simulink model "snap_adc5g_spec"  (R2019a)
settings: Solver=VariableStepDiscrete  StartTime=0.0  StopTime=10.0  RelTol=1e-3
undefined symbols (not defined in the file): pfb_coeff_gen_calc
libraries: xbsIndex_r4 x13965, casper_library_misc x80, casper_library_delays x43, xps_library x5, xbsReplacements_r4 x2, casper_library_communications x1
(part 75 of 152)

== system snap_adc5g_spec/fft_wideband_real/fft_biplex_real_4x/biplex_core/fft_stage_11/butterfly_direct/twiddle ==
  ai : Inport
  bi : Inport  Port=2
  sync_in : Inport  Port=3
  bus_convert : Subsystem  AncestorBlock=casper_library_bus/bus_convert  mask(bus_convert){n_bits_in=repmat(input_bit_width+coeff_bit_width+1, 1, n_inputs), bin_pt_in=(bin_pt_in+coeff_bit_width-1), cmplx=on, n_bits_out=input_bit_width+1, bin_pt_out=bin_pt_in, quantization=2, overflow=0, csp_latency=conv_latency, of=off, misc=on}
      mask prompts: n_bits_in "input bit widths"; bin_pt_in "input binary points"; cmplx "input complex"; n_bits_out "output bit widths"; bin_pt_out "output binary points"; quantization "quantization strategy (Truncate=0, Round  (unbiased: +/- Inf)=1, Round (unbiased: Even Values)=2)"; overflow "overflow strategy (Wrap=0, Saturate=1, Flag as error=2)"; csp_latency "latency"; of "overflow indication"; misc "misc support"
      mask help: Convert components of busses
      mask init: same as snap_adc5g_spec/fft_wideband_real/fft_direct/butterfly0_0/bus_convert
  bus_create : Subsystem  AncestorBlock=casper_library_flow_control/bus_create  mask(bus_create){inputNum=3}
      mask prompts: inputNum "Number of inputs:"
      mask init:
      | bus_create_init(gcb,...
      |     'inputNum', inputNum);
  bus_expand : Subsystem  AncestorBlock=casper_library_flow_control/bus_expand  mask(bus_expand){mode=divisions of arbitrary size, outputNum=1, outputWidth=[n_inputs*input_bit_width*2, 1+(n_inputs*input_bit_width*2)], outputBinaryPt=[0 0], outputArithmeticType=[0 0], show_format=off, outputToWorkspace=off, variablePrefix=out, outputToModelAsWell=on}
      mask prompts: outputNum "Number of outputs:"; outputWidth "Output width [msb ... lsb]:"; outputBinaryPt "Output binary point position [msb ... lsb]:"; outputArithmeticType "Output arithmetic type (ufix=0, fix=1, bool=2) [msb ... lsb]:"; show_format "Print format string?"; outputToWorkspace "Output to workspace?"; variablePrefix "Variable name prefix:"; outputToModelAsWell "Output to model as well?"
      mask help:
      | Expands a 'bus' made using a bus_create or Xilinx
      | concat block.
      | The input will be divided into the specified number
      | of outputs with the specified arithmetic types.
      | Divisions are made from most significant bit.
      mask init: same as snap_adc5g_spec/ss_adc/ctrl_split
      settings: AttributesFormatString=2 outputs
      mask TypeOptions mode: divisions of equal size | divisions of arbitrary size
      mask Callback mode: bus_expand_callback();
      mask Callback outputWidth: bus_expand_callback();
      mask Callback outputToWorkspace: bus_expand_callback();
  bus_expand1 : Subsystem  AncestorBlock=casper_library_flow_control/bus_expand  mask(bus_expand){mode=divisions of arbitrary size, outputNum=1, outputWidth=[1 72], outputBinaryPt=[0 0], outputArithmeticType=[2 0], show_format=off, outputToWorkspace=off, variablePrefix=out, outputToModelAsWell=on}
      mask prompts: outputNum "Number of outputs:"; outputWidth "Output width [msb ... lsb]:"; outputBinaryPt "Output binary point position [msb ... lsb]:"; outputArithmeticType "Output arithmetic type (ufix=0, fix=1, bool=2) [msb ... lsb]:"; show_format "Print format string?"; outputToWorkspace "Output to workspace?"; variablePrefix "Variable name prefix:"; outputToModelAsWell "Output to model as well?"
      mask help:
      | Expands a 'bus' made using a bus_create or Xilinx
      | concat block.
      | The input will be divided into the specified number
      | of outputs with the specified arithmetic types.
      | Divisions are made from most significant bit.
      mask init: same as snap_adc5g_spec/ss_adc/ctrl_split
      settings: AttributesFormatString=2 outputs
      mask TypeOptions mode: divisions of equal size | divisions of arbitrary size
      mask Callback mode: bus_expand_callback();
      mask Callback outputWidth: bus_expand_callback();
      mask Callback outputToWorkspace: bus_expand_callback();
  bus_mult : Subsystem  AncestorBlock=casper_library_bus/bus_mult  mask(bus_mult){n_bits_a=coeff_bit_width, bin_pt_a=coeff_bit_width-1, type_a=1, cmplx_a=on, n_bits_b=[18 18], bin_pt_b=bin_pt_in, type_b=1, cmplx_b=on, misc=on, floating_point=off, float_type=single, input_vec_a=1, input_vec_b=1, frac_width=24, exp_width=8, n_bits_out=input_bit_width+coeff_bit_width+1, bin_pt_out=(bin_pt_in+coeff_bit_width-1), type_out=1, quantization=0, overflow=0, mult_latency=mult_latency, add_latency=add_latency, conv_latency=0, max_fanout=max_fanout, fan_latency=2, multiplier_implementation=behavioral HDL, pipeline_cmult_en=off, pipeline_latency=0}
      mask prompts: n_bits_a "a input bit widths"; bin_pt_a "a input binary points"; type_a "a input type (Unsigned=0, Signed=1)"; cmplx_a "a input complex"; n_bits_b "b input bit widths"; bin_pt_b "b input binary points"; type_b "b input type (Unsigned=0, Signed=1)"; cmplx_b "b input complex"; misc "misc support"; floating_point "floating point"; float_type "float type"; input_vec_a "a input vector in bus"; input_vec_b "b input vector in bus"; frac_width "fraction width"; exp_width "exponent width"; n_bits_out "output bit widths"; bin_pt_out "output binary points"; type_out "output type (Unsigned=0, Signed=1)"; quantization "quantization strategy (Truncate=0, Round  (unbiased: +/- Inf)=1)"; overflow "overflow strategy (Wrap=0, Saturate=1, Flag as error=2)"; mult_latency "multiplier latency"; add_latency "adder latency"; conv_latency "convert latency"; max_fanout "limit fanout to ?"; fan_latency "fanout register latency"; multiplier_implementation "multiplier implementation"; pipeline_cmult_en "pipeline complex mult"; pipeline_latency "pipeline latency"
      mask help: Multiply components of two busses
      mask init: same as snap_adc5g_spec/fft_wideband_real/fft_direct/butterfly0_0/twiddle/bus_mult
      mask Callback floating_point:
      | onoff = get_param(gcb, 'floating_point');
      | if strcmp(onoff,'on')
      |     enable_fixpt = 'off';
      |     set_param_state(gcb, 'float_type', 'on')
      | 
      |     set_param_state(gcb, 'input_vec_a', 'on')
      |     set_param_state(gcb, 'input_vec_b', 'on')
      | 
      |     f_type = get_param(gcb, 'float_type');
      |     if strcmp(f_type,'custom')
      |         set_param_state(gcb, 'exp_width', 'on')
      |         set_param_state(gcb, 'frac_width', 'on')
      |     else
      |         set_param_state(gcb, 'exp_width', 'off')
      |         set_param_state(gcb, 'frac_width', 'off')
      |     end
      | 
      | else
      |     enable_fixpt = 'on';
      |     set_param_state(gcb, 'float_type', 'off')
      |     set_param_state(gcb, 'exp_width', 'off')
      |     set_param_state(gcb, 'frac_width', 'off')
      |     set_param_state(gcb, 'input_vec_a', 'off')
      |     set_param_state(gcb, 'input_vec_b', 'off')
      | end
      | 
      | set_param_state(gcb, 'n_bits_a', enable_fixpt)
      | set_param_state(gcb, 'bin_pt_a', enable_fixpt)
      | set_param_state(gcb, 'type_a', enable_fixpt)
      | set_param_state(gcb, 'n_bits_b', enable_fixpt)
      | set_param_state(gcb, 'bin_pt_b', enable_fixpt)
      | set_param_state(gcb, 'type_b', enable_fixpt)
      | 
      | set_param_state(gcb, 'n_bits_out', enable_fixpt)
      | set_param_state(gcb, 'bin_pt_out', enable_fixpt)
      | set_param_state(gcb, 'type_out', enable_fixpt)
      | set_param_state(gcb, 'quantization', enable_fixpt)
      | set_param_state(gcb, 'overflow', enable_fixpt)
      mask TypeOptions float_type: single | custom
      mask Callback float_type:
      | f_type = get_param(gcb, 'float_type');
      | if strcmp(f_type,'custom')
      |     set_param_state(gcb, 'exp_width', 'on')
      |     set_param_state(gcb, 'frac_width', 'on')
      | else
      |     set_param_state(gcb, 'exp_width', 'off')
      |     set_param_state(gcb, 'frac_width', 'off')
      | end
      mask TypeOptions multiplier_implementation: behavioral HDL | standard core | embedded multiplier core
      mask Callback pipeline_cmult_en:
      | pipeline_en = get_param(gcb, 'pipeline_cmult_en');
      | if strcmp(pipeline_en,'on')
      | 
      |     set_param_state(gcb, 'pipeline_latency', 'on')
      | else
      |     set_param_state(gcb, 'pipeline_latency', 'off')
      | end
  coeff_gen : Subsystem  AncestorBlock=casper_library_ffts_twiddle_coeff_gen/coeff_gen  mask(coeff_gen){FFTSize=FFTSize, Coeffs=[0 1 2 3 4 5 6 7 8 9 10 11 12 13 14 15 16 17 18 19 20 21 22 23 24 25 26 27 28 29 30 31 32 33 34 35 36 37 38 39 40 41 42 43 44 45 46 47 48 49 50 51 52 53 54 55 56 57 58 59 60 61 62 63 64 65 66 67 68 69 70 71 72 73 74 75 76 77 78 79 80 81 82 83 84 85 86 87 88 89 90 91 92 93 94 95 96 97 98 99 100 101 102 103 104 105 106 107 108 109 110 111 112 113 114 115 116 117 118 119 120 121 122 123 124 125 126 127 128 129 130 131 132 133 134 135 136 137 138 139 140 141 142 143 144 145 146 147 148 149 150 151 152 153 154 155 156 157 158 159 160 161 162 163 164 165 166 167 168 169 170 171 172 173 174 175 176 177 178 179 180 181 182 183 184 185 186 187 188 189 190 191 192 193 194 195 196 197 198 199 200 201 202 203 204 205 206 207 208 209 210 211 212 213 214 215 216 217 218 219 220 221 222 223 224 225 226 227 228 229 230 231 232 233 234 235 236 237 238 239 240 241 242 243 244 245 246 247 248 249 250 251 252 253 254 255 256 257 258 259 260 261 262 263 264 265 266 267 268 269 270 271 272 273 274 275 276 277 278 279 280 281 282 283 284 285 286 287 288 289 290 291 292 293 294 295 296 297 298 299 300 301 302 303 304 305 306 307 308 309 310 311 312 313 314 315 316 317 318 319 320 321 322 323 324 325 326 327 328 329 330 331 332 333 334 335 336 337 338 339 340 341 342 343 344 345 346 347 348 349 350 351 352 353 354 355 356 357 358 359 360 361 362 363 364 365 366 367 368 369 370 371 372 373 374 375 376 377 378 379 380 381 382 383 384 385 386 387 388 389 390 391 392 393 394 395 396 397 398 399 400 401 402 403 404 405 406 407 408 409 410 411 412 413 414 415 416 417 418 419 420 421 422 423 424 425 426 427 428 429 430 431 432 433 434 435 436 437 438 439 440 441 442 443 444 445 446 447 448 449 450 451 452 453 454 455 456 457 458 459 460 461 462 463 464 465 466 467 468 469 470 471 472 473 474 475 476 477 478 479 480 481 482 483 484 485 486 487 488 489 490 491 492 493 494 495 496 497 498 499 500 501 502 503 504 505 506 507 508 509 510 511 512 513 514 515 516 517 518 519 520 521 522 523 524 525 526 527 528 529 530 531 532 533 534 535 536 537 538 539 540 541 542 543 544 545 546 547 548 549 550 551 552 553 554 555 556 557 558 559 560 561 562 563 564 565 566 567 568 569 570 571 572 573 574 575 576 577 578 579 580 581 582 583 584 585 586 587 588 589 590 591 592 593 594 595 596 597 598 599 600 601 602 603 604 605 606 607 608 609 610 611 612 613 614 615 616 617 618 619 620 621 622 623 624 625 626 627 628 629 630 631 632 633 634 635 636 637 638 639 640 641 642 643 644 645 646 647 648 649 650 651 652 653 654 655 656 657 658 659 660 661 662 663 664 665 666 667 668 669 670 671 672 673 674 675 676 677 678 679 680 681 682 683 684 685 686 687 688 689 690 691 692 693 694 695 696 697 698 699 700 701 702 703 704 705 706 707 708 709 710 711 712 713 714 715 716 717 718 719 720 721 722 723 724 725 726 727 728 729 730 731 732 733 734 735 736 737 738 739 740 741 742 743 744 745 746 747 748 749 750 751 752 753 754 755 756 757 758 759 760 761 762 763 764 765 766 767 768 769 770 771 772 773 774 775 776 777 778 779 780 781 782 783 784 785 786 787 788 789 790 791 792 793 794 795 796 797 798 799 800 801 802 803 804 805 806 807 808 809 810 811 812 813 814 815 816 817 818 819 820 821 822 823 824 825 826 827 828 829 830 831 832 833 834 835 836 837 838 839 840 841 842 843 844 845 846 847 848 849 850 851 852 853 854 855 856 857 858 859 860 861 862 863 864 865 866 867 868 869 870 871 872 873 874 875 876 877 878 879 880 881 882 883 884 885 886 887 888 889 890 891 892 893 894 895 896 897 898 899 900 901 902 903 904 905 906 907 908 909 910 911 912 913 914 915 916 917 918 919 920 921 922 923 924 925 926 927 928 929 930 931 932 933 934 935 936 937 938 939 940 941 942 943 944 945 946 947 948 949 950 951 952 953 954 955 956 957 958 959 960 961 962 963 964 965 966 967 968 969 970 971 972 973 974 975 976 977 978 979 980 981 982 983 984 985 986 987 988 989 990 991 992 993 994 995 996 997 998 999 1000 1001 1002 1003 1004 1005 1006 1007 1008 1009 1010 1011 1012 1013 1014 1015 1016 1017 1018 1019 1020 1021 1022 1023], coeff_bit_width=coeff_bit_width, StepPeriod=StepPeriod, async=off, misc=on, floating_point=off, float_type=single, exp_width=8, frac_width=24, bram_latency=bram_latency, mult_latency=mult_latency, add_latency=add_latency, conv_latency=conv_latency, coeffs_bit_limit=coeffs_bit_limit, coeff_sharing=on, coeff_decimation=on, coeff_generation=off, cal_bits=cal_bits, n_bits_rotation=n_bits_rotation, quantization=Round  (unbiased: Even Values)}
      mask prompts: FFTSize "fft size (2^?)"; Coeffs "Coefficients"; coeff_bit_width "Coefficient Bit Width:"; StepPeriod "Step Period: (2^?)"; async "asynchronous operation"; misc "misc port"; floating_point "floating point"; exp_width "exponential width"; frac_width "fractional width"; bram_latency "BRAM latency"; mult_latency "Multiplier latency"; add_latency "Adder latency"; conv_latency "Convert latency"; coeffs_bit_limit "Number bits above which to store stage's coefficients in BRAM (2^? bits)"; coeff_sharing "BRAM sharing in coeff storage"; coeff_decimation "Store a fraction of coeff factors where useful"; coeff_generation "Generate coeffs with multipliers where useful"; cal_bits "Number calibration locations when generating coeffs (2^?)"; n_bits_rotation "Rotation vector resolution"; quantization "Quantization strategy"
      mask help:
      | Generates a sequence of complex coefficients for use in generating twiddle
      | factors for FFTs.
      mask init: same as snap_adc5g_spec/fft_wideband_real/fft_direct/butterfly0_0/twiddle/coeff_gen
      settings: AttributesFormatString=1024 @ (18,17)
      mask Callback floating_point:
      | onoff = get_param(gcb, 'floating_point');
      | if strcmp(onoff,'on')
      |     enable_fixpt = 'off'
      |     set_param_state(gcb, 'float_type', 'on')
      | 
      |     f_type = get_param(gcb, 'float_type')
      |     if strcmp(f_type,'custom')
      |         set_param_state(gcb, 'exp_width', 'on')
      |         set_param_state(gcb, 'frac_width', 'on')
      |     else
      |         set_param_state(gcb, 'exp_width', 'off')
      |         set_param_state(gcb, 'frac_width', 'off')
      |     end
      | 
      | 
      | else
      |     enable_fixpt = 'on'
      |     set_param_state(gcb, 'float_type', 'off')
      |     set_param_state(gcb, 'exp_width', 'off')
      |     set_param_state(gcb, 'frac_width', 'off')
      | end
      mask TypeOptions float_type: single | custom
      mask Callback float_type:
      | f_type = get_param(gcb, 'float_type')
      | if strcmp(f_type,'custom')
      |     set_param_state(gcb, 'exp_width', 'on')
      |     set_param_state(gcb, 'frac_width', 'on')
      | else
      |     set_param_state(gcb, 'exp_width', 'off')
      |     set_param_state(gcb, 'frac_width', 'off')
      | end
      mask TypeOptions quantization: Truncate | Round  (unbiased: +/- Inf) | Round  (unbiased: Even Values)
      mask DialogControl ParameterTabVar0 Prompt: basic
      mask DialogControl ParameterTabVar01 Prompt: latency
      mask DialogControl ParameterTabVar012 Prompt: implementation
  ao : Outport
  bwo : Outport  Port=2
  sync_out : Outport  Port=3
  wires:
  bi/1 -> bus_create/1(in1)
  sync_in/1 -> bus_create/2(in2), coeff_gen/1(rst)
  ai/1 -> bus_create/3(in3)
  bus_create/1(bus_out) -> coeff_gen/2(misci)
  coeff_gen/2(misco) -> bus_expand/1(bus_in)
  coeff_gen/1(w) -> bus_mult/1(a)
  bus_expand/2(lsb_out1) -> bus_mult/3(misci)
  bus_expand/1(msb_out2) -> bus_mult/2(b)
  bus_mult/1(a*b) -> bus_convert/1(din)
  bus_mult/2(misco) -> bus_convert/2(misci)
  bus_convert/1(dout) -> bwo/1
  bus_convert/2(misco) -> bus_expand1/1(bus_in)
  bus_expand1/1(msb_out2) -> sync_out/1
  bus_expand1/2(lsb_out1) -> ao/1

== system snap_adc5g_spec/fft_wideband_real/fft_biplex_real_4x/biplex_core/fft_stage_11/delay0/din_expand ==
  bus_in : Inport
  reinterpret1 : xbsIndex_r4/Reinterpret  force_arith_type=on  arith_type=Unsigned  force_bin_pt=on  bin_pt=0  block_type=reinterpret
  reinterpret2 : xbsIndex_r4/Reinterpret  force_arith_type=on  arith_type=Unsigned  force_bin_pt=on  bin_pt=0  block_type=reinterpret
  slice1 : xbsIndex_r4/Slice  nbits=36  boolean_output=off  mode=Upper Bit Location + Width  bit1=-36  base1=MSB of Input  bit0=0  base0=LSB of Input  dbl_ovrd=off  block_type=slice
  slice2 : xbsIndex_r4/Slice  nbits=36  boolean_output=off  mode=Upper Bit Location + Width  bit1=0  base1=MSB of Input  bit0=0  base0=LSB of Input  dbl_ovrd=off  block_type=slice
  msb_out2 : Outport
  lsb_out1 : Outport  Port=2
  wires:
  bus_in/1 -> slice2/1, slice1/1
  slice2/1 -> reinterpret2/1
  reinterpret2/1 -> msb_out2/1
  slice1/1 -> reinterpret1/1
  reinterpret1/1 -> lsb_out1/1

== system snap_adc5g_spec/fft_wideband_real/fft_biplex_real_4x/biplex_core/fft_stage_11/delay0/dout_compress ==
  in1 : Inport
  in2 : Inport  Port=2
  concatenate : xbsIndex_r4/Concat  num_inputs=2  dbl_ovrd=off  block_type=concat
  reinterpret1 : xbsIndex_r4/Reinterpret  force_arith_type=on  arith_type=Unsigned  force_bin_pt=on  bin_pt=0  block_type=reinterpret
      settings: infoedit="Changes signal type without altering the binary representation.   You can changed the signal between signed and unsigned, and relocate the binary point.<br><br>Hardware notes: In hardware this block costs nothing.<br><br>Example:  Suppose the input is 6 bits wide, signed, with 2 fractional bits, and the output is forced to unsigned with 0 fractional bits.  Then an input of -2.0 (1110.00 in binary 2's complement) becomes an output of 56 (111000 in binary)."
  reinterpret2 : xbsIndex_r4/Reinterpret  force_arith_type=on  arith_type=Unsigned  force_bin_pt=on  bin_pt=0  block_type=reinterpret
      settings: infoedit="Changes signal type without altering the binary representation.   You can changed the signal between signed and unsigned, and relocate the binary point.<br><br>Hardware notes: In hardware this block costs nothing.<br><br>Example:  Suppose the input is 6 bits wide, signed, with 2 fractional bits, and the output is forced to unsigned with 0 fractional bits.  Then an input of -2.0 (1110.00 in binary 2's complement) becomes an output of 56 (111000 in binary)."
  bus_out : Outport
  wires:
  concatenate/1 -> bus_out/1
  in1/1 -> reinterpret1/1
  reinterpret1/1 -> concatenate/1
  in2/1 -> reinterpret2/1
  reinterpret2/1 -> concatenate/2

== system snap_adc5g_spec/fft_wideband_real/fft_biplex_real_4x/biplex_core/fft_stage_11/delay1/din_expand ==
  bus_in : Inport
  reinterpret1 : xbsIndex_r4/Reinterpret  force_arith_type=on  arith_type=Unsigned  force_bin_pt=on  bin_pt=0  block_type=reinterpret
  reinterpret2 : xbsIndex_r4/Reinterpret  force_arith_type=on  arith_type=Unsigned  force_bin_pt=on  bin_pt=0  block_type=reinterpret
  slice1 : xbsIndex_r4/Slice  nbits=36  boolean_output=off  mode=Upper Bit Location + Width  bit1=-36  base1=MSB of Input  bit0=0  base0=LSB of Input  dbl_ovrd=off  block_type=slice
  slice2 : xbsIndex_r4/Slice  nbits=36  boolean_output=off  mode=Upper Bit Location + Width  bit1=0  base1=MSB of Input  bit0=0  base0=LSB of Input  dbl_ovrd=off  block_type=slice
  msb_out2 : Outport
  lsb_out1 : Outport  Port=2
  wires:
  bus_in/1 -> slice2/1, slice1/1
  slice2/1 -> reinterpret2/1
  reinterpret2/1 -> msb_out2/1
  slice1/1 -> reinterpret1/1
  reinterpret1/1 -> lsb_out1/1

== system snap_adc5g_spec/fft_wideband_real/fft_biplex_real_4x/biplex_core/fft_stage_11/delay1/dout_compress ==
  in1 : Inport
  in2 : Inport  Port=2
  concatenate : xbsIndex_r4/Concat  num_inputs=2  dbl_ovrd=off  block_type=concat
  reinterpret1 : xbsIndex_r4/Reinterpret  force_arith_type=on  arith_type=Unsigned  force_bin_pt=on  bin_pt=0  block_type=reinterpret
      settings: infoedit="Changes signal type without altering the binary representation.   You can changed the signal between signed and unsigned, and relocate the binary point.<br><br>Hardware notes: In hardware this block costs nothing.<br><br>Example:  Suppose the input is 6 bits wide, signed, with 2 fractional bits, and the output is forced to unsigned with 0 fractional bits.  Then an input of -2.0 (1110.00 in binary 2's complement) becomes an output of 56 (111000 in binary)."
  reinterpret2 : xbsIndex_r4/Reinterpret  force_arith_type=on  arith_type=Unsigned  force_bin_pt=on  bin_pt=0  block_type=reinterpret
      settings: infoedit="Changes signal type without altering the binary representation.   You can changed the signal between signed and unsigned, and relocate the binary point.<br><br>Hardware notes: In hardware this block costs nothing.<br><br>Example:  Suppose the input is 6 bits wide, signed, with 2 fractional bits, and the output is forced to unsigned with 0 fractional bits.  Then an input of -2.0 (1110.00 in binary 2's complement) becomes an output of 56 (111000 in binary)."
  bus_out : Outport
  wires:
  concatenate/1 -> bus_out/1
  in1/1 -> reinterpret1/1
  reinterpret1/1 -> concatenate/1
  in2/1 -> reinterpret2/1
  reinterpret2/1 -> concatenate/2

== system snap_adc5g_spec/fft_wideband_real/fft_biplex_real_4x/biplex_core/fft_stage_2/butterfly_direct/bus_add ==
  a : Inport
  b : Inport  Port=2
  a_debus : Subsystem  AncestorBlock=casper_library_flow_control/bus_expand  mask(bus_expand){mode=divisions of arbitrary size, outputNum=1, outputWidth=[18  18  18  18], outputBinaryPt=[17  17  17  17], outputArithmeticType=[1  1  1  1], show_format=on, outputToWorkspace=off, variablePrefix=, outputToModelAsWell=on}
      mask prompts: outputNum "Number of outputs:"; outputWidth "Output width [msb ... lsb]:"; outputBinaryPt "Output binary point position [msb ... lsb]:"; outputArithmeticType "Output arithmetic type (ufix=0, fix=1, bool=2) [msb ... lsb]:"; show_format "Print format string?"; outputToWorkspace "Output to workspace?"; variablePrefix "Variable name prefix:"; outputToModelAsWell "Output to model as well?"
      mask help:
      | Expands a 'bus' made using a bus_create or Xilinx
      | concat block.
      | The input will be divided into the specified number
      | of outputs with the specified arithmetic types.
      | Divisions are made from most significant bit.
      mask init: same as snap_adc5g_spec/ss_adc/ctrl_split
      settings: AttributesFormatString=4 outputs: f18.17,f18.17,f18.17,f18.17,
      mask TypeOptions mode: divisions of equal size | divisions of arbitrary size
      mask Callback mode: bus_expand_callback();
      mask Callback outputWidth: bus_expand_callback();
      mask Callback outputToWorkspace: bus_expand_callback();
  addsub{1..4} (4 alike) : xbsIndex_r4/AddSub  mode=Addition  use_carryin=off  use_carryout=off  en=off  latency=1  precision=User Defined  arith_type="Signed  (2's comp)"  n_bits=19  bin_pt=17  quantization=Truncate  overflow=Wrap  use_behavioral_HDL=on  hw_selection=Fabric  pipelined=on  dbl_ovrd=off  block_type=addsub
  b_debus : Subsystem  AncestorBlock=casper_library_flow_control/bus_expand  mask(bus_expand){mode=divisions of arbitrary size, outputNum=1, outputWidth=[18  18  18  18], outputBinaryPt=[17  17  17  17], outputArithmeticType=[1  1  1  1], show_format=on, outputToWorkspace=off, variablePrefix=, outputToModelAsWell=on}
      mask prompts: outputNum "Number of outputs:"; outputWidth "Output width [msb ... lsb]:"; outputBinaryPt "Output binary point position [msb ... lsb]:"; outputArithmeticType "Output arithmetic type (ufix=0, fix=1, bool=2) [msb ... lsb]:"; show_format "Print format string?"; outputToWorkspace "Output to workspace?"; variablePrefix "Variable name prefix:"; outputToModelAsWell "Output to model as well?"
      mask help:
      | Expands a 'bus' made using a bus_create or Xilinx
      | concat block.
      | The input will be divided into the specified number
      | of outputs with the specified arithmetic types.
      | Divisions are made from most significant bit.
      mask init: same as snap_adc5g_spec/ss_adc/ctrl_split
      settings: AttributesFormatString=4 outputs: f18.17,f18.17,f18.17,f18.17,
      mask TypeOptions mode: divisions of equal size | divisions of arbitrary size
      mask Callback mode: bus_expand_callback();
      mask Callback outputWidth: bus_expand_callback();
      mask Callback outputToWorkspace: bus_expand_callback();
  op_bussify : Subsystem  AncestorBlock=casper_library_flow_control/bus_create  mask(bus_create){inputNum=4}
      mask prompts: inputNum "Number of inputs:"
      mask init:
      | bus_create_init(gcb,...
      |     'inputNum', inputNum);
  dout : Outport
  wires:
  a/1 -> a_debus/1(bus_in)
  b/1 -> b_debus/1(bus_in)
  a_debus/1(msb_out4) -> addsub1/1
  b_debus/1(msb_out4) -> addsub1/2
  a_debus/2(out3) -> addsub2/1
  b_debus/2(out3) -> addsub2/2
  a_debus/3(out2) -> addsub3/1
  b_debus/3(out2) -> addsub3/2
  a_debus/4(lsb_out1) -> addsub4/1
  b_debus/4(lsb_out1) -> addsub4/2
  addsub1/1 -> op_bussify/1(in1)
  addsub2/1 -> op_bussify/2(in2)
  addsub3/1 -> op_bussify/3(in3)
  addsub4/1 -> op_bussify/4(in4)
  op_bussify/1(bus_out) -> dout/1

== system snap_adc5g_spec/fft_wideband_real/fft_biplex_real_4x/biplex_core/fft_stage_2/butterfly_direct/bus_convert ==
  din : Inport
  bussify : Subsystem  AncestorBlock=casper_library_flow_control/bus_create  mask(bus_create){inputNum=8}
      mask prompts: inputNum "Number of inputs:"
      mask init:
      | bus_create_init(gcb,...
      |     'inputNum', inputNum);
  conv1 : Subsystem  AncestorBlock=casper_library_misc/convert_of  mask(convert_of){bit_width_i=20, binary_point_i=18, bit_width_o=18, binary_point_o=17, csp_latency=1, overflow=Wrap, quantization=Round  (unbiased: even values)}
      mask prompts: bit_width_i "Bit Width In"; binary_point_i "Binary Point In"; bit_width_o "Bit Width Out"; binary_point_o "Binary Point Out"; csp_latency "Latency"; overflow "Overflow Behaviour"; quantization "Quantization Behaviour"
      mask help:
      | Converts from one 2's complement bit-width
      | and/or binary point position to another.
      | Includes underflow/overflow indicator.
      mask init: same as snap_adc5g_spec/fft_wideband_real/fft_direct/butterfly0_0/bus_convert/conv1
      settings: AttributesFormatString=[20,18]->[18,17]
      mask TypeOptions overflow: Wrap | Saturate | Error
      mask TypeOptions quantization: Truncate | Round  (unbiased: +/- Inf) | Round  (unbiased: even values)
  conv2 : Subsystem  AncestorBlock=casper_library_misc/convert_of  mask(convert_of){bit_width_i=20, binary_point_i=18, bit_width_o=18, binary_point_o=17, csp_latency=1, overflow=Wrap, quantization=Round  (unbiased: even values)}
      mask prompts: bit_width_i "Bit Width In"; binary_point_i "Binary Point In"; bit_width_o "Bit Width Out"; binary_point_o "Binary Point Out"; csp_latency "Latency"; overflow "Overflow Behaviour"; quantization "Quantization Behaviour"
      mask help:
      | Converts from one 2's complement bit-width
      | and/or binary point position to another.
      | Includes underflow/overflow indicator.
      mask init: same as snap_adc5g_spec/fft_wideband_real/fft_direct/butterfly0_0/bus_convert/conv1
      settings: AttributesFormatString=[20,18]->[18,17]
      mask TypeOptions overflow: Wrap | Saturate | Error
      mask TypeOptions quantization: Truncate | Round  (unbiased: +/- Inf) | Round  (unbiased: even values)
  conv3 : Subsystem  AncestorBlock=casper_library_misc/convert_of  mask(convert_of){bit_width_i=20, binary_point_i=18, bit_width_o=18, binary_point_o=17, csp_latency=1, overflow=Wrap, quantization=Round  (unbiased: even values)}
      mask prompts: bit_width_i "Bit Width In"; binary_point_i "Binary Point In"; bit_width_o "Bit Width Out"; binary_point_o "Binary Point Out"; csp_latency "Latency"; overflow "Overflow Behaviour"; quantization "Quantization Behaviour"
      mask help:
      | Converts from one 2's complement bit-width
      | and/or binary point position to another.
      | Includes underflow/overflow indicator.
      mask init: same as snap_adc5g_spec/fft_wideband_real/fft_direct/butterfly0_0/bus_convert/conv1
      settings: AttributesFormatString=[20,18]->[18,17]
      mask TypeOptions overflow: Wrap | Saturate | Error
      mask TypeOptions quantization: Truncate | Round  (unbiased: +/- Inf) | Round  (unbiased: even values)
  conv4 : Subsystem  AncestorBlock=casper_library_misc/convert_of  mask(convert_of){bit_width_i=20, binary_point_i=18, bit_width_o=18, binary_point_o=17, csp_latency=1, overflow=Wrap, quantization=Round  (unbiased: even values)}
      mask prompts: bit_width_i "Bit Width In"; binary_point_i "Binary Point In"; bit_width_o "Bit Width Out"; binary_point_o "Binary Point Out"; csp_latency "Latency"; overflow "Overflow Behaviour"; quantization "Quantization Behaviour"
      mask help:
      | Converts from one 2's complement bit-width
      | and/or binary point position to another.
      | Includes underflow/overflow indicator.
      mask init: same as snap_adc5g_spec/fft_wideband_real/fft_direct/butterfly0_0/bus_convert/conv1
      settings: AttributesFormatString=[20,18]->[18,17]
      mask TypeOptions overflow: Wrap | Saturate | Error
      mask TypeOptions quantization: Truncate | Round  (unbiased: +/- Inf) | Round  (unbiased: even values)
  conv5 : Subsystem  AncestorBlock=casper_library_misc/convert_of  mask(convert_of){bit_width_i=20, binary_point_i=18, bit_width_o=18, binary_point_o=17, csp_latency=1, overflow=Wrap, quantization=Round  (unbiased: even values)}
      mask prompts: bit_width_i "Bit Width In"; binary_point_i "Binary Point In"; bit_width_o "Bit Width Out"; binary_point_o "Binary Point Out"; csp_latency "Latency"; overflow "Overflow Behaviour"; quantization "Quantization Behaviour"
      mask help:
      | Converts from one 2's complement bit-width
      | and/or binary point position to another.
      | Includes underflow/overflow indicator.
      mask init: same as snap_adc5g_spec/fft_wideband_real/fft_direct/butterfly0_0/bus_convert/conv1
      settings: AttributesFormatString=[20,18]->[18,17]
      mask TypeOptions overflow: Wrap | Saturate | Error
      mask TypeOptions quantization: Truncate | Round  (unbiased: +/- Inf) | Round  (unbiased: even values)
  conv6 : Subsystem  AncestorBlock=casper_library_misc/convert_of  mask(convert_of){bit_width_i=20, binary_point_i=18, bit_width_o=18, binary_point_o=17, csp_latency=1, overflow=Wrap, quantization=Round  (unbiased: even values)}
      mask prompts: bit_width_i "Bit Width In"; binary_point_i "Binary Point In"; bit_width_o "Bit Width Out"; binary_point_o "Binary Point Out"; csp_latency "Latency"; overflow "Overflow Behaviour"; quantization "Quantization Behaviour"
      mask help:
      | Converts from one 2's complement bit-width
      | and/or binary point position to another.
      | Includes underflow/overflow indicator.
      mask init: same as snap_adc5g_spec/fft_wideband_real/fft_direct/butterfly0_0/bus_convert/conv1
      settings: AttributesFormatString=[20,18]->[18,17]
      mask TypeOptions overflow: Wrap | Saturate | Error
      mask TypeOptions quantization: Truncate | Round  (unbiased: +/- Inf) | Round  (unbiased: even values)
  conv7 : Subsystem  AncestorBlock=casper_library_misc/convert_of  mask(convert_of){bit_width_i=20, binary_point_i=18, bit_width_o=18, binary_point_o=17, csp_latency=1, overflow=Wrap, quantization=Round  (unbiased: even values)}
      mask prompts: bit_width_i "Bit Width In"; binary_point_i "Binary Point In"; bit_width_o "Bit Width Out"; binary_point_o "Binary Point Out"; csp_latency "Latency"; overflow "Overflow Behaviour"; quantization "Quantization Behaviour"
      mask help:
      | Converts from one 2's complement bit-width
      | and/or binary point position to another.
      | Includes underflow/overflow indicator.
      mask init: same as snap_adc5g_spec/fft_wideband_real/fft_direct/butterfly0_0/bus_convert/conv1
      settings: AttributesFormatString=[20,18]->[18,17]
      mask TypeOptions overflow: Wrap | Saturate | Error
      mask TypeOptions quantization: Truncate | Round  (unbiased: +/- Inf) | Round  (unbiased: even values)
  conv8 : Subsystem  AncestorBlock=casper_library_misc/convert_of  mask(convert_of){bit_width_i=20, binary_point_i=18, bit_width_o=18, binary_point_o=17, csp_latency=1, overflow=Wrap, quantization=Round  (unbiased: even values)}
      mask prompts: bit_width_i "Bit Width In"; binary_point_i "Binary Point In"; bit_width_o "Bit Width Out"; binary_point_o "Binary Point Out"; csp_latency "Latency"; overflow "Overflow Behaviour"; quantization "Quantization Behaviour"
      mask help:
      | Converts from one 2's complement bit-width
      | and/or binary point position to another.
      | Includes underflow/overflow indicator.
      mask init: same as snap_adc5g_spec/fft_wideband_real/fft_direct/butterfly0_0/bus_convert/conv1
      settings: AttributesFormatString=[20,18]->[18,17]
      mask TypeOptions overflow: Wrap | Saturate | Error
      mask TypeOptions quantization: Truncate | Round  (unbiased: +/- Inf) | Round  (unbiased: even values)
  debus : Subsystem  AncestorBlock=casper_library_flow_control/bus_expand  mask(bus_expand){mode=divisions of arbitrary size, outputNum=1, outputWidth=[20 20 20 20 20 20 20 20], outputBinaryPt=[18 18 18 18 18 18 18 18], outputArithmeticType=[1 1 1 1 1 1 1 1], show_format=on, outputToWorkspace=off, variablePrefix=, outputToModelAsWell=on}
      mask prompts: outputNum "Number of outputs:"; outputWidth "Output width [msb ... lsb]:"; outputBinaryPt "Output binary point position [msb ... lsb]:"; outputArithmeticType "Output arithmetic type (ufix=0, fix=1, bool=2) [msb ... lsb]:"; show_format "Print format string?"; outputToWorkspace "Output to workspace?"; variablePrefix "Variable name prefix:"; outputToModelAsWell "Output to model as well?"
      mask help:
      | Expands a 'bus' made using a bus_create or Xilinx
      | concat block.
      | The input will be divided into the specified number
      | of outputs with the specified arithmetic types.
      | Divisions are made from most significant bit.
      mask init: same as snap_adc5g_spec/ss_adc/ctrl_split
      settings: AttributesFormatString=8 outputs: f20.18,f20.18,f20.18,f20.18,f20.18,f20.18,f20.18,f20.18,
      mask TypeOptions mode: divisions of equal size | divisions of arbitrary size
      mask Callback mode: bus_expand_callback();
      mask Callback outputWidth: bus_expand_callback();
      mask Callback outputToWorkspace: bus_expand_callback();
  of_bussify : Subsystem  AncestorBlock=casper_library_flow_control/bus_create  mask(bus_create){inputNum=8}
      mask prompts: inputNum "Number of inputs:"
      mask init:
      | bus_create_init(gcb,...
      |     'inputNum', inputNum);
  dout : Outport
  overflow : Outport  Port=2
  wires:
  din/1 -> debus/1(bus_in)
  debus/1(msb_out8) -> conv1/1(din)
  debus/2(out7) -> conv2/1(din)
  debus/3(out6) -> conv3/1(din)
  debus/4(out5) -> conv4/1(din)
  debus/5(out4) -> conv5/1(din)
  debus/6(out3) -> conv6/1(din)
  debus/7(out2) -> conv7/1(din)
  debus/8(lsb_out1) -> conv8/1(din)
  conv1/1(dout) -> bussify/1(in1)
  conv2/1(dout) -> bussify/2(in2)
  conv3/1(dout) -> bussify/3(in3)
  conv4/1(dout) -> bussify/4(in4)
  conv5/1(dout) -> bussify/5(in5)
  conv6/1(dout) -> bussify/6(in6)
  conv7/1(dout) -> bussify/7(in7)
  conv8/1(dout) -> bussify/8(in8)
  conv1/2(of) -> of_bussify/1(in1)
  conv2/2(of) -> of_bussify/2(in2)
  conv3/2(of) -> of_bussify/3(in3)
  conv4/2(of) -> of_bussify/4(in4)
  conv5/2(of) -> of_bussify/5(in5)
  conv6/2(of) -> of_bussify/6(in6)
  conv7/2(of) -> of_bussify/7(in7)
  conv8/2(of) -> of_bussify/8(in8)
  bussify/1(bus_out) -> dout/1
  of_bussify/1(bus_out) -> overflow/1

== system snap_adc5g_spec/fft_wideband_real/fft_biplex_real_4x/biplex_core/fft_stage_2/butterfly_direct/bus_expand ==
  bus_in : Inport
  reinterpret1 : xbsIndex_r4/Reinterpret  force_arith_type=on  arith_type=Unsigned  force_bin_pt=on  bin_pt=0  block_type=reinterpret
  reinterpret2 : xbsIndex_r4/Reinterpret  force_arith_type=on  arith_type=Unsigned  force_bin_pt=on  bin_pt=0  block_type=reinterpret
  slice1 : xbsIndex_r4/Slice  nbits=72  boolean_output=off  mode=Upper Bit Location + Width  bit1=-72  base1=MSB of Input  bit0=0  base0=LSB of Input  dbl_ovrd=off  block_type=slice
  slice2 : xbsIndex_r4/Slice  nbits=72  boolean_output=off  mode=Upper Bit Location + Width  bit1=0  base1=MSB of Input  bit0=0  base0=LSB of Input  dbl_ovrd=off  block_type=slice
  msb_out2 : Outport
  lsb_out1 : Outport  Port=2
  wires:
  bus_in/1 -> slice2/1, slice1/1
  slice2/1 -> reinterpret2/1
  reinterpret2/1 -> msb_out2/1
  slice1/1 -> reinterpret1/1
  reinterpret1/1 -> lsb_out1/1

== system snap_adc5g_spec/fft_wideband_real/fft_biplex_real_4x/biplex_core/fft_stage_2/butterfly_direct/bus_norm0 ==
  din : Inport
  bussify : Subsystem  AncestorBlock=casper_library_flow_control/bus_create  mask(bus_create){inputNum=8}
      mask prompts: inputNum "Number of inputs:"
      mask init:
      | bus_create_init(gcb,...
      |     'inputNum', inputNum);
  conv{1..8} (8 alike) : xbsIndex_r4/Convert  gui_display_data_type=Fixed-point  arith_type="Signed  (2's comp)"  n_bits=20  bin_pt=18  float_type=Single  exp_bits=8  fraction_bits=24  quantization=Truncate  overflow=Wrap  en=off  latency=0  pipeline=on  dbl_ovrd=off  block_type=convert
  debus : Subsystem  AncestorBlock=casper_library_flow_control/bus_expand  mask(bus_expand){mode=divisions of arbitrary size, outputNum=1, outputWidth=[19 19 19 19 19 19 19 19], outputBinaryPt=[17 17 17 17 17 17 17 17], outputArithmeticType=[1 1 1 1 1 1 1 1], show_format=on, outputToWorkspace=off, variablePrefix=, outputToModelAsWell=on}
      mask prompts: outputNum "Number of outputs:"; outputWidth "Output width [msb ... lsb]:"; outputBinaryPt "Output binary point position [msb ... lsb]:"; outputArithmeticType "Output arithmetic type (ufix=0, fix=1, bool=2) [msb ... lsb]:"; show_format "Print format string?"; outputToWorkspace "Output to workspace?"; variablePrefix "Variable name prefix:"; outputToModelAsWell "Output to model as well?"
      mask help:
      | Expands a 'bus' made using a bus_create or Xilinx
      | concat block.
      | The input will be divided into the specified number
      | of outputs with the specified arithmetic types.
      | Divisions are made from most significant bit.
      mask init: same as snap_adc5g_spec/ss_adc/ctrl_split
      settings: AttributesFormatString=8 outputs: f19.17,f19.17,f19.17,f19.17,f19.17,f19.17,f19.17,f19.17,
      mask TypeOptions mode: divisions of equal size | divisions of arbitrary size
      mask Callback mode: bus_expand_callback();
      mask Callback outputWidth: bus_expand_callback();
      mask Callback outputToWorkspace: bus_expand_callback();
  dout : Outport
  wires:
  din/1 -> debus/1(bus_in)
  debus/1(msb_out8) -> conv1/1
  debus/2(out7) -> conv2/1
  debus/3(out6) -> conv3/1
  debus/4(out5) -> conv4/1
  debus/5(out4) -> conv5/1
  debus/6(out3) -> conv6/1
  debus/7(out2) -> conv7/1
  debus/8(lsb_out1) -> conv8/1
  conv1/1 -> bussify/1(in1)
  conv2/1 -> bussify/2(in2)
  conv3/1 -> bussify/3(in3)
  conv4/1 -> bussify/4(in4)
  conv5/1 -> bussify/5(in5)
  conv6/1 -> bussify/6(in6)
  conv7/1 -> bussify/7(in7)
  conv8/1 -> bussify/8(in8)
  bussify/1(bus_out) -> dout/1
